simulink model "TestSupervisorFSM_RX"  (R2023b)
settings: Solver=FixedStepDiscrete  StartTime=0.0  StopTime=inf  FixedStep=0.001  RelTol=1e-3  EnableMultiTasking=on
model workspace (MAT data in the model file):
  Command = 1
  SelectedControlMode = 0
  State = 0
  pid_kp = 1
undefined symbols (not defined in the file): CANErrorTypes, ControlModes, MCControlModes
libraries: eeStairGenerator x7
settings Model: DataDictionary=EmbeddedBoardDD.sldd  Creator=vvasco  LastModifiedBy=upattacini
settings SolverCC: AlgebraicLoopSolver=TrustRegion  AutoInsertRateTranBlk=on
settings DataIOCC: LimitDataPoints=on
settings OptimizationCC: ReuseModelBlockBuffer=off  LifeSpan=inf
settings DebuggingCC: ParameterPrecisionLossMsg=none  UnconnectedInputMsg=warning  UnconnectedOutputMsg=warning  UnconnectedLineMsg=warning  AllowSymbolicDim=off  SFUnexpectedBacktrackingDiag=warning  SFNoUnconditionalDefaultTransitionDiag=warning  SFExecutionAtInitializationDiag=none  ArithmeticOperatorsInVariantConditions=warning
settings ModelReferenceCC: EnableRefExpFcnMdlSchedulingChecks=on
settings SFSimCC: SimUseLocalCustomCode=off  CustomCodeUndefinedFunction=UseInterfaceOnly
settings RTWCC: RTWUseLocalCustomCode=off  DLArmComputeVersion=19.05
settings CodeAppCC: StateflowObjectComments=on
settings GRTTargetCC: TargetLangStandard=C89/C90 (ANSI)
settings ConfigComp: CovMetricSettings=dw  CovSaveCumulativeToWorkspaceVar=on  CovSaveSingleToWorkspaceVar=on  CovExternalEMLEnable=off

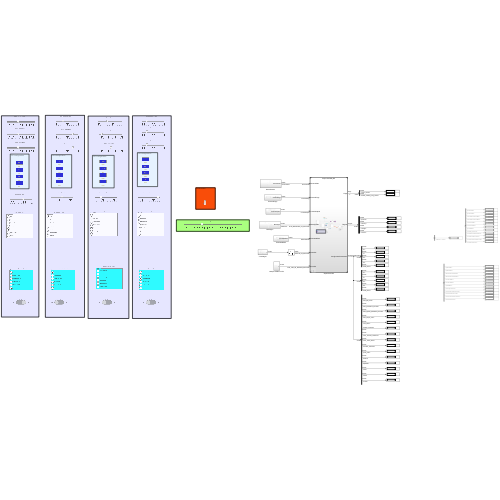
[thumbnail: Simulink's stored preview of the top-level diagram]
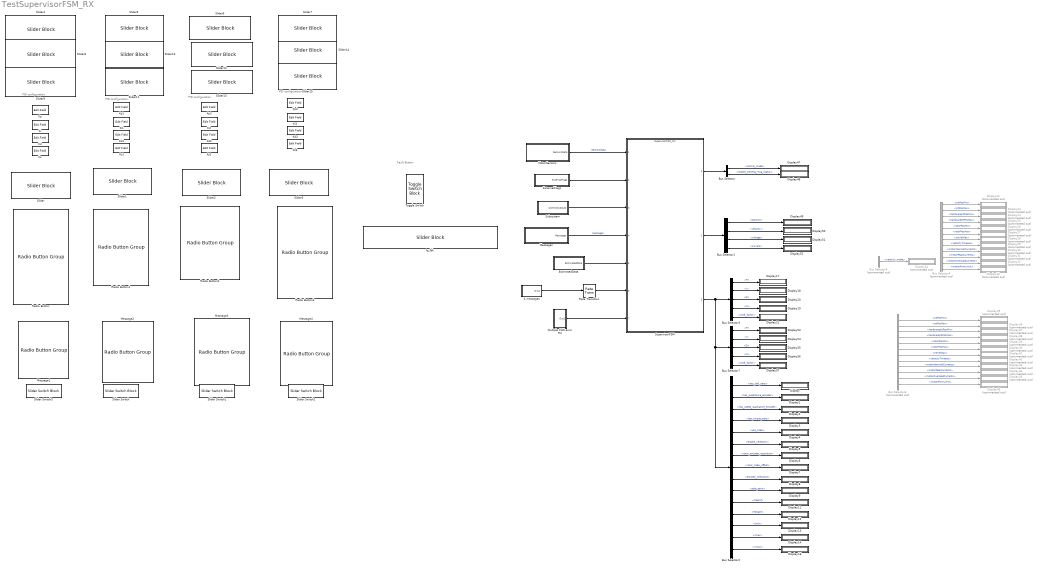
== system TestSupervisorFSM_RX ==
  note: Fault Button
  note: PID configuration
  note: PID configuration
  note: PID configuration
  note: PID configuration
  4 messages : Subsystem
  Bus Selector : BusSelector  OutputSignals=control_mode,enable_sending_msg_status
  Bus Selector1 : BusSelector  OutputSignals=jointpositions.position,jointvelocities.velocity,motorvoltage.voltage,motorcurrent.current
  Bus Selector2 : BusSelector  OutputSignals=motorconfig.has_hall_sens,motorconfig.has_quadrature_encoder,motorconfig.has_speed_quadrature_encoder,motorconfig.has_torque_sens,motorconfig.use_index,motorconfig.enable_verbosity,motorconfig.rotor_encoder_resolution,motorconfig.rotor_index_offset,motorconfig.encoder_tolerance,motorconfig.pole_pairs,motorconfig.Kbemf,motorconfig.Rphase,motorconfig.Imin,motorconfig.Imax,motorconfig.Vmax
  Bus Selector3 : BusSelector  OutputSignals=CurLoopPID.P,CurLoopPID.I,CurLoopPID.D,CurLoopPID.N,CurLoopPID.shift_factor
  Bus Selector4 : BusSelector  Commented=on  OutputSignals=thresholds.jntPosMin,thresholds.jntPosMax,thresholds.hardwareJntPosMin,thresholds.hardwareJntPosMax,thresholds.rotorPosMin,thresholds.rotorPosMax,thresholds.jntVelMax,thresholds.velocityTimeout,thresholds.motorNominalCurrents,thresholds.motorPeakCurrents,thresholds.motorOverloadCurrents,thresholds.motorPwmLimit
  Bus Selector5 : BusSelector  Commented=on  OutputSignals=estimationconfig.velocity_mode
  Bus Selector6 : BusSelector  Commented=on  OutputSignals=thresholds.jntPosMin,thresholds.jntPosMax,thresholds.hardwareJntPosMin,thresholds.hardwareJntPosMax,thresholds.rotorPosMin,thresholds.rotorPosMax,thresholds.jntVelMax,thresholds.velocityTimeout,thresholds.motorNominalCurrents,thresholds.motorPeakCurrents,thresholds.motorOverloadCurrents,thresholds.motorPwmLimit
  Bus Selector7 : BusSelector  OutputSignals=VelLoopPID.P,VelLoopPID.I,VelLoopPID.D,VelLoopPID.N,VelLoopPID.shift_factor
  Display{,1..9,11..14,16..21,47..57} (31 alike) : Display
  Display{22..46} (25 alike) : Display  Commented=on
  EstimatedData : Subsystem
  ExternalFlags : Subsystem
  Iq_fbk : SliderBlock  ScaleMax=20
  Kd{,1..3} (4 alike) : EditField  LabelPosition=Hide  ShowInitialText=on  Alignment=Center
  Ki{,1..3} (4 alike) : EditField  LabelPosition=Hide  ShowInitialText=on  Alignment=Center
  Kp{,1..3} (4 alike) : EditField  LabelPosition=Hide  ShowInitialText=on  Alignment=Center
  Ks{,1..3} (4 alike) : EditField  LabelPosition=Hide  ShowInitialText=on  Alignment=Center
  Message1 : RadioButtonGroup  SelectedLabel=Set MotorConfig  ButtonGroupName=Group
      settings: Values={{'Set control mode', 'Set current limits', 'Set desired targets', 'Set current PID', 'Set Velocity PID', 'Set MotorConfig'}, [0 1 2 3 4 5]}
  Message2 : RadioButtonGroup  SelectedLabel=Set control mode  ButtonGroupName=Group
      settings: Values={{'Set control mode', 'Set current limits', 'Set desired target', 'Set current PID', 'Set velocity PID', 'Set MotorConfig'}, [0 1 2 3 4 5]}
  Message3 : RadioButtonGroup  SelectedLabel=Set desired target  ButtonGroupName=Group
      settings: Values={{'Set control mode', 'Set current limits', 'Set desired target', 'Set current PID', 'Set velocity PID', 'Set MotorConfig'}, [0 1 2 3 4 5]}
  Message4 : RadioButtonGroup  SelectedLabel=Set desired target  ButtonGroupName=Group
      settings: Values={{'Set control mode', 'Set current limits', 'Set desired target', 'Set current PID', 'Set Velocity PID', 'Set MotorConfig'}, [0 1 2 3 4 5]}
  Messages : Subsystem
  MotorSensors : Subsystem
  Multiple CAN error RX : Subsystem
  Radio Button : RadioButtonGroup  SelectedLabel=Current  ButtonGroupName=Control Mode  UseEnumeratedDataType=on  EnumeratedDataType=MCControlModes
      settings: Values={{'Idle', 'OpenLoop', 'SpeedVoltage', 'SpeedCurrent', 'Current', 'NotConfigured', 'HWFault'}, [0 80 10 11 6 176 160]}
  Radio Button1 : RadioButtonGroup  SelectedLabel=Idle  ButtonGroupName=Control Mode  UseEnumeratedDataType=on  EnumeratedDataType=MCControlModes
      settings: Values={{'Idle', 'OpenLoop', 'SpeedVoltage', 'SpeedCurrent', 'Current', 'NotConfigured', 'HWFault'}, [0 80 10 11 6 176 160]}
  Radio Button2 : RadioButtonGroup  SelectedLabel=Current  ButtonGroupName=Control Mode  UseEnumeratedDataType=on  EnumeratedDataType=MCControlModes
      settings: Values={{'Idle', 'OpenLoop', 'SpeedVoltage', 'SpeedCurrent', 'Current', 'NotConfigured', 'HWFault'}, [0 80 10 11 6 176 160]}
  Radio Button3 : RadioButtonGroup  SelectedLabel=Current  ButtonGroupName=Control Mode  UseEnumeratedDataType=on  EnumeratedDataType=MCControlModes
      settings: Values={{'Idle', 'OpenLoop', 'SpeedVoltage', 'SpeedCurrent', 'Current', 'NotConfigured', 'HWFault'}, [0 80 10 11 6 176 160]}
  Rate Transition : RateTransition  Deterministic=off  OutPortSampleTimeOpt=Inherit
  Slider{,1..3} (4 alike) : SliderBlock  ScaleMin=10  ScaleMax=20
  Slider Switch{,1..3} (4 alike) : SliderSwitchBlock
      settings: Values={{'Off', 'On'}, [0 1]}
  Slider{4..15} (12 alike) : SliderBlock  ScaleMax=20
  Subsystem : Subsystem
  SupervisorFSM : ModelReference  ModelNameDialog=SupervisorFSM_RX.slx  SimulationMode=Normal  ModelReferenceVersion=7.4
  Toggle Switch : ToggleSwitchBlock  LabelPosition=Hide
      settings: Values={{'Off', 'On'}, [0 1]}
  wires:
  SupervisorFSM/2 -> Bus Selector1/1
  MotorSensors/1(SensorsData) -> SupervisorFSM/1  "SensorsData"
  SupervisorFSM/1 -> Bus Selector/1
  Bus Selector/1 -> Display47/1  "<control_mode>"
  Subsystem/1(ControlOutputs) -> SupervisorFSM/3
  ExternalFlags/1(externalFlags) -> SupervisorFSM/2
  Bus Selector/2 -> Display48/1  "<enable_sending_msg_status>"
  Bus Selector1/1 -> Display49/1  "<position>"
  Bus Selector1/2 -> Display50/1  "<velocity>"
  Bus Selector1/3 -> Display51/1  "<voltage>"
  Bus Selector1/4 -> Display52/1  "<current>"
  Rate Transition/1 -> SupervisorFSM/6
  Messages/1(Messages) -> SupervisorFSM/4  "Messages"
  EstimatedData/1(EstimatedData) -> SupervisorFSM/5
  Multiple CAN error RX/1(Out1) -> SupervisorFSM/7
  4 messages/1(Out1) -> Rate Transition/1
  Bus Selector2/1 -> Display/1  "<has_hall_sens>"
  Bus Selector2/2 -> Display1/1  "<has_quadrature_encoder>"
  Bus Selector2/3 -> Display2/1  "<has_speed_quadrature_encoder>"
  Bus Selector2/4 -> Display3/1  "<has_torque_sens>"
  Bus Selector2/5 -> Display4/1  "<use_index>"
  Bus Selector2/6 -> Display5/1  "<enable_verbosity>"
  Bus Selector2/7 -> Display6/1  "<rotor_encoder_resolution>"
  Bus Selector2/8 -> Display7/1  "<rotor_index_offset>"
  Bus Selector2/9 -> Display8/1  "<encoder_tolerance>"
  Bus Selector2/10 -> Display9/1  "<pole_pairs>"
  Bus Selector2/11 -> Display11/1  "<Kbemf>"
  Bus Selector2/12 -> Display12/1  "<Rphase>"
  Bus Selector2/13 -> Display13/1  "<Imin>"
  Bus Selector2/14 -> Display14/1  "<Imax>"
  Bus Selector3/1 -> Display17/1  "<P>"
  Bus Selector3/2 -> Display18/1  "<I>"
  Bus Selector3/3 -> Display20/1  "<D>"
  Bus Selector3/4 -> Display19/1  "<N>"
  Bus Selector3/5 -> Display21/1  "<shift_factor>"
  Bus Selector4/1 -> Display22/1  "<jntPosMin>"
  Bus Selector4/2 -> Display23/1  "<jntPosMax>"
  Bus Selector4/3 -> Display24/1  "<hardwareJntPosMin>"
  Bus Selector4/4 -> Display25/1  "<hardwareJntPosMax>"
  Bus Selector4/5 -> Display26/1  "<rotorPosMin>"
  Bus Selector4/6 -> Display27/1  "<rotorPosMax>"
  Bus Selector4/7 -> Display28/1  "<jntVelMax>"
  Bus Selector4/8 -> Display29/1  "<velocityTimeout>"
  Bus Selector4/9 -> Display30/1  "<motorNominalCurrents>"
  Bus Selector4/10 -> Display31/1  "<motorPeakCurrents>"
  Bus Selector4/11 -> Display32/1  "<motorOverloadCurrents>"
  Bus Selector4/12 -> Display33/1  "<motorPwmLimit>"
  Bus Selector5/1 -> Display34/1  "<velocity_mode>"
  Bus Selector6/1 -> Display35/1  "<jntPosMin>"
  Bus Selector6/2 -> Display36/1  "<jntPosMax>"
  Bus Selector6/3 -> Display37/1  "<hardwareJntPosMin>"
  Bus Selector6/4 -> Display38/1  "<hardwareJntPosMax>"
  Bus Selector6/5 -> Display39/1  "<rotorPosMin>"
  Bus Selector6/6 -> Display40/1  "<rotorPosMax>"
  Bus Selector6/7 -> Display41/1  "<jntVelMax>"
  Bus Selector6/8 -> Display42/1  "<velocityTimeout>"
  Bus Selector6/9 -> Display43/1  "<motorNominalCurrents>"
  Bus Selector6/10 -> Display44/1  "<motorPeakCurrents>"
  Bus Selector6/11 -> Display45/1  "<motorOverloadCurrents>"
  Bus Selector6/12 -> Display46/1  "<motorPwmLimit>"
  SupervisorFSM/3 -> Bus Selector2/1, Bus Selector7/1, Bus Selector3/1
  Bus Selector7/1 -> Display53/1  "<P>"
  Bus Selector7/2 -> Display54/1  "<I>"
  Bus Selector7/3 -> Display55/1  "<D>"
  Bus Selector7/4 -> Display56/1  "<N>"
  Bus Selector7/5 -> Display57/1  "<shift_factor>"
  Bus Selector2/15 -> Display16/1  "<Vmax>"

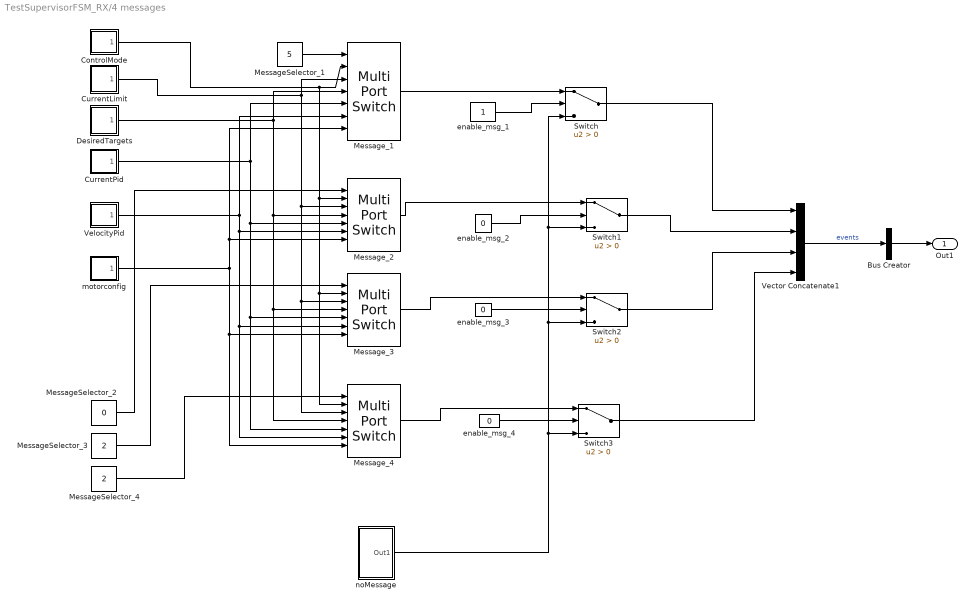
== system TestSupervisorFSM_RX/4 messages ==
  Bus Creator : BusCreator  Inputs=1  OutDataTypeStr=Bus: BUS_STATUS_RX_MULTIPLE  NonVirtualBus=on
      settings: InheritFromInputs=off
  ControlMode : Subsystem
  CurrentLimit : Subsystem
  CurrentPid : Subsystem
  DesiredTargets : Subsystem
  MessageSelector_1 : Constant  Value=5
  MessageSelector_2 : Constant  Value=0
  MessageSelector_3 : Constant  Value=2
  MessageSelector_4 : Constant  Value=2
  Message_{1..4} (4 alike) : MultiPortSwitch  DataPortOrder=Zero-based contiguous  Inputs=6  zeroidx=on  SaturateOnIntegerOverflow=off  InputSameDT=off
  Switch{,1..3} (4 alike) : Switch  Criteria=u2 > Threshold  SaturateOnIntegerOverflow=off  InputSameDT=off
  Vector Concatenate1 : Concatenate  NumInputs=4
  VelocityPid : Subsystem
  enable_msg_1 : Constant
  enable_msg_2 : Constant  Value=0
  enable_msg_3 : Constant  Value=0
  enable_msg_4 : Constant  Value=0
  motorconfig : Subsystem
  noMessage : Subsystem
  Out1 : Outport  OutDataTypeStr=Bus: BUS_STATUS_RX_MULTIPLE
  wires:
  MessageSelector_1/1 -> Message_1/1
  ControlMode/1(Out1) -> Message_4/2, Message_3/2, Message_2/2, Message_1/2
  CurrentPid/1(Out1) -> Message_2/5, Message_4/5, Message_3/5, Message_1/5
  MessageSelector_3/1 -> Message_3/1
  Vector Concatenate1/1 -> Bus Creator/1  "events"
  MessageSelector_4/1 -> Message_4/1
  DesiredTargets/1(Out1) -> Message_4/4, Message_3/4, Message_2/4, Message_1/4
  CurrentLimit/1(Out1) -> Message_4/3, Message_3/3, Message_2/3, Message_1/3
  MessageSelector_2/1 -> Message_2/1
  Bus Creator/1 -> Out1/1
  noMessage/1(Out1) -> Switch3/3, Switch1/3, Switch/3, Switch2/3
  enable_msg_1/1 -> Switch/2
  Message_1/1 -> Switch/1
  Message_2/1 -> Switch1/1
  enable_msg_2/1 -> Switch1/2
  Message_3/1 -> Switch2/1
  enable_msg_3/1 -> Switch2/2
  enable_msg_4/1 -> Switch3/2
  Message_4/1 -> Switch3/1
  Switch/1 -> Vector Concatenate1/1
  Switch1/1 -> Vector Concatenate1/2
  Switch2/1 -> Vector Concatenate1/3
  Switch3/1 -> Vector Concatenate1/4
  VelocityPid/1(Out1) -> Message_2/6, Message_4/6, Message_3/6, Message_1/6
  motorconfig/1(Out1) -> Message_4/7, Message_3/7, Message_2/7, Message_1/7

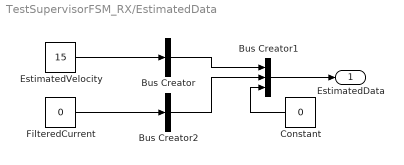
== system TestSupervisorFSM_RX/EstimatedData ==
  Bus Creator : BusCreator  Inputs=1  OutDataTypeStr=Bus: JointVelocities  NonVirtualBus=on
      settings: InheritFromInputs=off
  Bus Creator1 : BusCreator  Inputs=3  OutDataTypeStr=Bus: EstimatedData  NonVirtualBus=on
      settings: InheritFromInputs=off
  Bus Creator2 : BusCreator  Inputs=1  OutDataTypeStr=Bus: MotorCurrent  NonVirtualBus=on
      settings: InheritFromInputs=off
  Constant : Constant  Value=0  OutDataTypeStr=Bus: MotorTemperature
  EstimatedVelocity : Constant  Value=15  OutDataTypeStr=single
  FilteredCurrent : Constant  Value=0  OutDataTypeStr=single
  EstimatedData : Outport
  wires:
  EstimatedVelocity/1 -> Bus Creator/1
  Bus Creator1/1 -> EstimatedData/1
  Bus Creator/1 -> Bus Creator1/1
  FilteredCurrent/1 -> Bus Creator2/1
  Bus Creator2/1 -> Bus Creator1/2
  Constant/1 -> Bus Creator1/3

== system TestSupervisorFSM_RX/ExternalFlags ==
  Constant : Constant  Value=logical(0)  OutDataTypeStr=boolean
  ExternalFlags : BusCreator  Inputs=1  OutDataTypeStr=Bus: ExternalFlags
  externalFlags : Outport
  wires:
  Constant/1 -> ExternalFlags/1  "fault_button"
  ExternalFlags/1 -> externalFlags/1

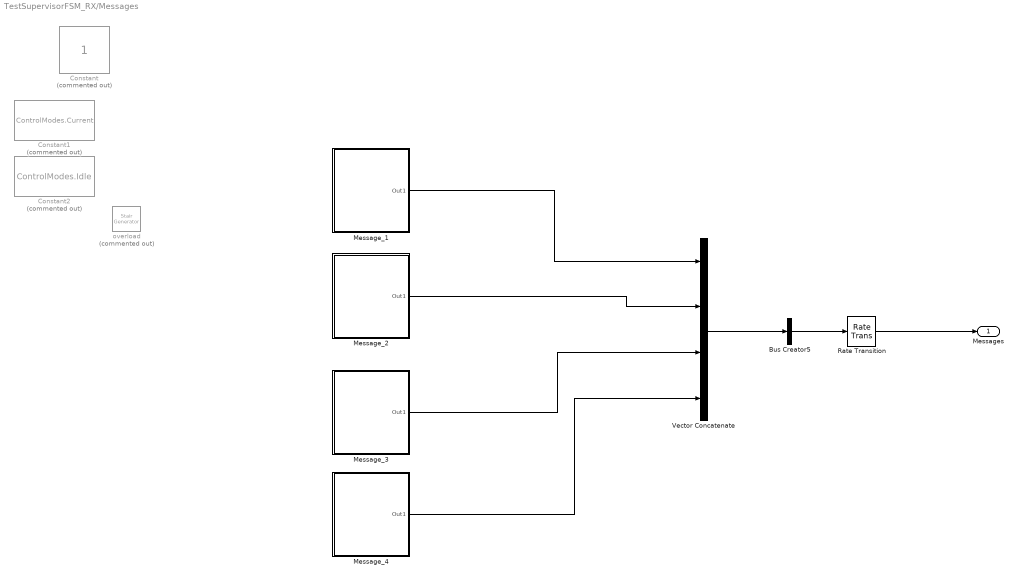
== system TestSupervisorFSM_RX/Messages ==
  Bus Creator5 : BusCreator  Inputs=1  OutDataTypeStr=Bus: BUS_MESSAGES_RX_MULTIPLE  NonVirtualBus=on
      settings: InheritFromInputs=off
  Constant : Constant  Commented=on  OutDataTypeStr=Enum: ControlModes
  Constant1 : Constant  Commented=on  Value=ControlModes.Current  OutDataTypeStr=Enum: ControlModes
  Constant2 : Constant  Commented=on  Value=ControlModes.Idle  OutDataTypeStr=Enum: ControlModes
  Message_1 : Subsystem
  Message_2 : Subsystem
  Message_3 : Subsystem
  Message_4 : Subsystem
  Rate Transition : RateTransition  Deterministic=off  OutPortSampleTimeOpt=Inherit
  Vector Concatenate : Concatenate  NumInputs=4
  overload : eeStairGenerator/Stair Generator  Commented=on  LabelModeActiveChoice=Discrete  TimeInput=[0 0.1 0.2 0.3 0.4 0.5 0.6 0.7 0.8 0.9]  AmplitudeInput=[5 0 5 1 1 1 1 1 1 1]  SampleTime=0.1  RepeatPattern=off  OutDataTypeStr=uint16
  Messages : Outport
  wires:
  Rate Transition/1 -> Messages/1
  Vector Concatenate/1 -> Bus Creator5/1
  Message_1/1(Out1) -> Vector Concatenate/1
  Message_2/1(Out1) -> Vector Concatenate/2
  Message_3/1(Out1) -> Vector Concatenate/3
  Message_4/1(Out1) -> Vector Concatenate/4
  Bus Creator5/1 -> Rate Transition/1

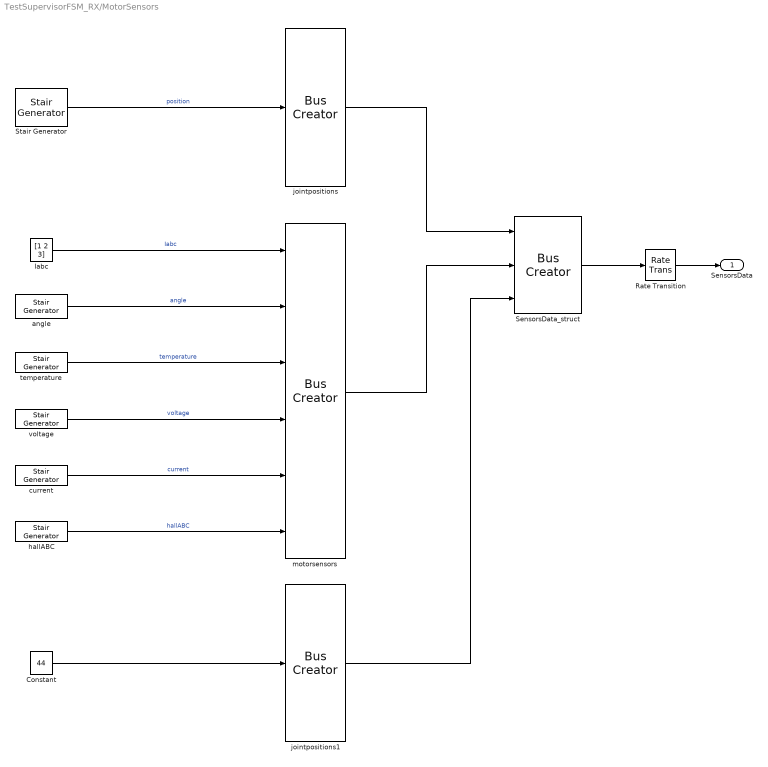
== system TestSupervisorFSM_RX/MotorSensors ==
  Constant : Constant  Value=44  OutDataTypeStr=single
  Iabc : Constant  Value=[1 2 3]  OutDataTypeStr=single
  Rate Transition : RateTransition  Deterministic=off  OutPortSampleTimeOpt=Inherit
  SensorsData_struct : BusCreator  Inputs=3  OutDataTypeStr=Bus: SensorsData
      settings: InheritFromInputs=off
  Stair Generator : eeStairGenerator/Stair Generator  LabelModeActiveChoice=Discrete  TimeInput=[0.1 0.2 0.3 0.4 0.5 0.6 0.7 0.8 0.9 1 1.1 1.2 1.3 ]  AmplitudeInput=[20 23 26 29 32 35 38 41 39 36 30 25 20]  SampleTime=0.1  RepeatPattern=on  OutDataTypeStr=single
  angle : eeStairGenerator/Stair Generator  LabelModeActiveChoice=Discrete  TimeInput=[0 1 2 3 4 5 6 7 8 9]  AmplitudeInput=[0 1 6 6 6 1 1 1 2 2]  SampleTime=0.1  RepeatPattern=off  OutDataTypeStr=single
  current : eeStairGenerator/Stair Generator  LabelModeActiveChoice=Discrete  TimeInput=[0 0.1 0.2 0.3 0.4 0.5 0.6 0.7 0.8 0.9]  AmplitudeInput=[16 10 15 12 10 16 12 16 18 17]  SampleTime=0.1  RepeatPattern=on  OutDataTypeStr=single
  hallABC : eeStairGenerator/Stair Generator  LabelModeActiveChoice=Discrete  TimeInput=[0 0.1 0.2 0.3 0.4 0.5 0.6 0.7 0.8 0.9]  AmplitudeInput=[6 3 5 2 0 6 6 6 6 6]  SampleTime=0.1  RepeatPattern=off  OutDataTypeStr=uint8
  jointpositions : BusCreator  Inputs=1  OutDataTypeStr=Bus: JointPositions
      settings: InheritFromInputs=off
  jointpositions1 : BusCreator  Inputs=1  OutDataTypeStr=Bus: SupplyVoltage
      settings: InheritFromInputs=off
  motorsensors : BusCreator  Inputs=6  OutDataTypeStr=Bus: MotorSensors
      settings: InheritFromInputs=off
  temperature : eeStairGenerator/Stair Generator  LabelModeActiveChoice=Discrete  TimeInput=[0 1 2 3 4 5 6 7 8 9]  AmplitudeInput=[2 2 2 9 9 9 9 9 9 2]  SampleTime=0.1  RepeatPattern=off  OutDataTypeStr=single
  voltage : eeStairGenerator/Stair Generator  LabelModeActiveChoice=Discrete  TimeInput=[0 1 2 3 4 5 6 7 8 9]./10  AmplitudeInput=[2 3 3 3 3 3 2 2 2 2]  SampleTime=0.1  RepeatPattern=on  OutDataTypeStr=single
  SensorsData : Outport  OutDataTypeStr=Bus: SensorsData
  wires:
  motorsensors/1 -> SensorsData_struct/2
  voltage/1 -> motorsensors/4  "voltage"
  angle/1 -> motorsensors/2  "angle"
  temperature/1 -> motorsensors/3  "temperature"
  current/1 -> motorsensors/5  "current"
  Iabc/1 -> motorsensors/1  "Iabc"
  hallABC/1 -> motorsensors/6  "hallABC"
  SensorsData_struct/1 -> Rate Transition/1
  Stair Generator/1 -> jointpositions/1  "position"
  jointpositions/1 -> SensorsData_struct/1
  Rate Transition/1 -> SensorsData/1
  jointpositions1/1 -> SensorsData_struct/3
  Constant/1 -> jointpositions1/1

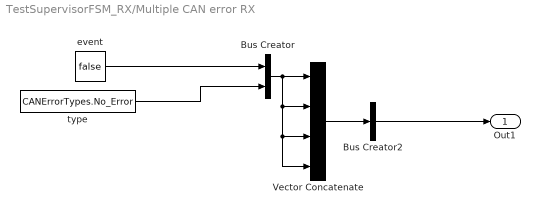
== system TestSupervisorFSM_RX/Multiple CAN error RX ==
  Bus Creator : BusCreator  Inputs=2  OutDataTypeStr=Bus: BUS_CAN_RX_ERRORS  NonVirtualBus=on
      settings: InheritFromInputs=off
  Bus Creator2 : BusCreator  Inputs=1  OutDataTypeStr=Bus: BUS_CAN_RX_ERRORS_MULTIPLE  NonVirtualBus=on
      settings: InheritFromInputs=off
  Vector Concatenate : Concatenate  NumInputs=4
  event : Constant  Value=false  OutDataTypeStr=boolean
  type : Constant  Value=CANErrorTypes.No_Error  OutDataTypeStr=Enum: CANErrorTypes
  Out1 : Outport
  wires:
  Bus Creator/1 -> Vector Concatenate/4, Vector Concatenate/3, Vector Concatenate/2, Vector Concatenate/1
  event/1 -> Bus Creator/1
  type/1 -> Bus Creator/2
  Vector Concatenate/1 -> Bus Creator2/1
  Bus Creator2/1 -> Out1/1

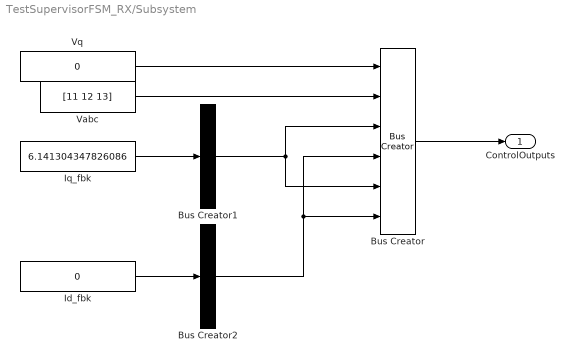
== system TestSupervisorFSM_RX/Subsystem ==
  Bus Creator : BusCreator  Inputs=6  OutDataTypeStr=Bus: ControlOutputs
      settings: InheritFromInputs=off
  Bus Creator1 : BusCreator  Inputs=1  OutDataTypeStr=Bus: MotorCurrent
      settings: InheritFromInputs=off
  Bus Creator2 : BusCreator  Inputs=1  OutDataTypeStr=Bus: MotorCurrent
      settings: InheritFromInputs=off
  Id_fbk : Constant  Value=0  OutDataTypeStr=single
  Iq_fbk : Constant  Value=6.141304347826086  OutDataTypeStr=single
  Vabc : Constant  Value=[11 12 13]  OutDataTypeStr=single
  Vq : Constant  Value=0  OutDataTypeStr=single
  ControlOutputs : Outport  OutDataTypeStr=Bus: ControlOutputs
  wires:
  Iq_fbk/1 -> Bus Creator1/1
  Bus Creator/1 -> ControlOutputs/1
  Bus Creator1/1 -> Bus Creator/5, Bus Creator/3
  Vabc/1 -> Bus Creator/2
  Vq/1 -> Bus Creator/1
  Bus Creator2/1 -> Bus Creator/6, Bus Creator/4
  Id_fbk/1 -> Bus Creator2/1

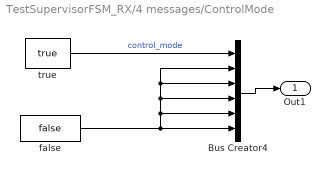
== system TestSupervisorFSM_RX/4 messages/ControlMode ==
  Bus Creator4 : BusCreator  Inputs=6  OutDataTypeStr=Bus: BUS_STATUS_RX  NonVirtualBus=on
      settings: InheritFromInputs=off
  false : Constant  Value=false  OutDataTypeStr=boolean
  true : Constant  Value=true  OutDataTypeStr=boolean
  Out1 : Outport  OutDataTypeStr=Bus: BUS_STATUS_RX
  wires:
  true/1 -> Bus Creator4/1  "control_mode"
  false/1 -> Bus Creator4/6, Bus Creator4/2, Bus Creator4/3, Bus Creator4/4, Bus Creator4/5
  Bus Creator4/1 -> Out1/1

== system TestSupervisorFSM_RX/4 messages/CurrentLimit ==
  Bus Creator5 : BusCreator  Inputs=6  OutDataTypeStr=Bus: BUS_STATUS_RX  NonVirtualBus=on
      settings: InheritFromInputs=off
  false1 : Constant  Value=false  OutDataTypeStr=boolean
  true1 : Constant  Value=true  OutDataTypeStr=boolean
  Out1 : Outport  OutDataTypeStr=Bus: BUS_STATUS_RX
  wires:
  false1/1 -> Bus Creator5/6, Bus Creator5/5, Bus Creator5/1, Bus Creator5/3, Bus Creator5/4
  true1/1 -> Bus Creator5/2
  Bus Creator5/1 -> Out1/1

== system TestSupervisorFSM_RX/4 messages/CurrentPid ==
  Bus Creator7 : BusCreator  Inputs=6  OutDataTypeStr=Bus: BUS_STATUS_RX  NonVirtualBus=on
      settings: InheritFromInputs=off
  false3 : Constant  Value=false  OutDataTypeStr=boolean
  true3 : Constant  Value=true  OutDataTypeStr=boolean
  Out1 : Outport  OutDataTypeStr=Bus: BUS_STATUS_RX
  wires:
  true3/1 -> Bus Creator7/4  "control_mode"
  false3/1 -> Bus Creator7/6, Bus Creator7/5, Bus Creator7/3, Bus Creator7/2, Bus Creator7/1
  Bus Creator7/1 -> Out1/1

== system TestSupervisorFSM_RX/4 messages/DesiredTargets ==
  Bus Creator6 : BusCreator  Inputs=6  OutDataTypeStr=Bus: BUS_STATUS_RX  NonVirtualBus=on
      settings: InheritFromInputs=off
  false2 : Constant  Value=false  OutDataTypeStr=boolean
  true2 : Constant  Value=true  OutDataTypeStr=boolean
  Out1 : Outport  OutDataTypeStr=Bus: BUS_STATUS_RX
  wires:
  true2/1 -> Bus Creator6/3  "control_mode"
  false2/1 -> Bus Creator6/6, Bus Creator6/5, Bus Creator6/2, Bus Creator6/1, Bus Creator6/4
  Bus Creator6/1 -> Out1/1

== system TestSupervisorFSM_RX/4 messages/VelocityPid ==
  Bus Creator7 : BusCreator  Inputs=6  OutDataTypeStr=Bus: BUS_STATUS_RX  NonVirtualBus=on
      settings: InheritFromInputs=off
  false3 : Constant  Value=false  OutDataTypeStr=boolean
  true3 : Constant  Value=true  OutDataTypeStr=boolean
  Out1 : Outport  OutDataTypeStr=Bus: BUS_STATUS_RX
  wires:
  true3/1 -> Bus Creator7/5  "control_mode"
  false3/1 -> Bus Creator7/3, Bus Creator7/6, Bus Creator7/4, Bus Creator7/2, Bus Creator7/1
  Bus Creator7/1 -> Out1/1

== system TestSupervisorFSM_RX/4 messages/motorconfig ==
  Bus Creator7 : BusCreator  Inputs=6  OutDataTypeStr=Bus: BUS_STATUS_RX  NonVirtualBus=on
      settings: InheritFromInputs=off
  false3 : Constant  Value=false  OutDataTypeStr=boolean
  true3 : Constant  Value=true  OutDataTypeStr=boolean
  Out1 : Outport  OutDataTypeStr=Bus: BUS_STATUS_RX
  wires:
  true3/1 -> Bus Creator7/6  "control_mode"
  false3/1 -> Bus Creator7/3, Bus Creator7/5, Bus Creator7/4, Bus Creator7/2, Bus Creator7/1
  Bus Creator7/1 -> Out1/1

== system TestSupervisorFSM_RX/4 messages/noMessage ==
  Bus Creator : BusCreator  Inputs=6  OutDataTypeStr=Bus: BUS_STATUS_RX  NonVirtualBus=on
      settings: InheritFromInputs=off
  Constant : Constant  Value=false
  Out1 : Outport
  wires:
  Constant/1 -> Bus Creator/6, Bus Creator/5, Bus Creator/4, Bus Creator/3, Bus Creator/2, Bus Creator/1
  Bus Creator/1 -> Out1/1

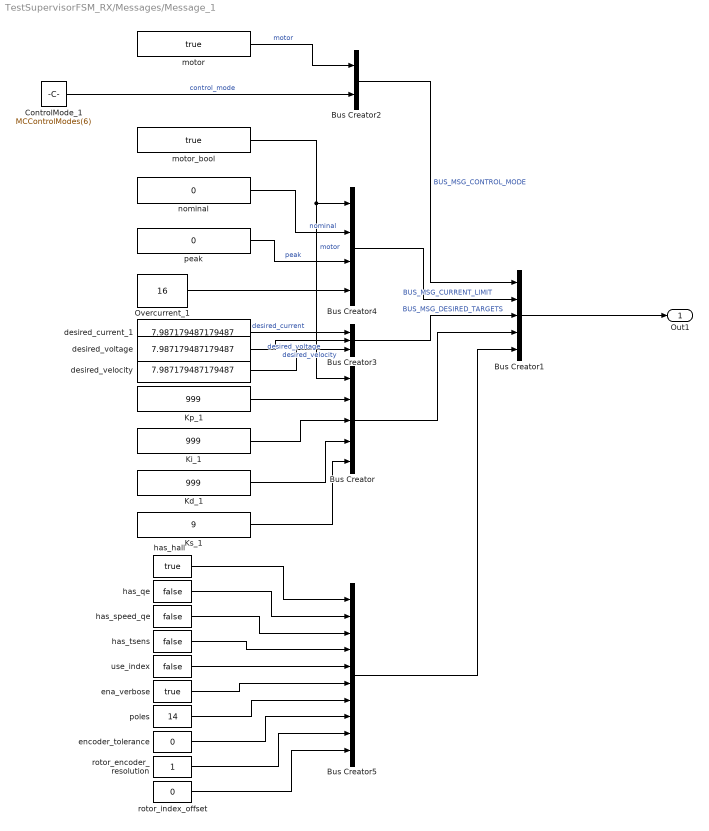
== system TestSupervisorFSM_RX/Messages/Message_1 ==
  Bus Creator : BusCreator  Inputs=5  OutDataTypeStr=Bus: BUS_MSG_PID  NonVirtualBus=on
      settings: InheritFromInputs=off
  Bus Creator1 : BusCreator  Inputs=5  OutDataTypeStr=Bus: BUS_MESSAGES_RX  NonVirtualBus=on
      settings: InheritFromInputs=off
  Bus Creator2 : BusCreator  Inputs=2  OutDataTypeStr=Bus: BUS_MSG_CONTROL_MODE  NonVirtualBus=on
      settings: InheritFromInputs=off
  Bus Creator3 : BusCreator  Inputs=3  OutDataTypeStr=Bus: BUS_MSG_DESIRED_TARGETS  NonVirtualBus=on
      settings: InheritFromInputs=off
  Bus Creator4 : BusCreator  Inputs=4  OutDataTypeStr=Bus: BUS_MSG_CURRENT_LIMIT  NonVirtualBus=on
      settings: InheritFromInputs=off
  Bus Creator5 : BusCreator  Inputs=10  OutDataTypeStr=Bus: BUS_MSG_MOTOR_CONFIG  NonVirtualBus=on
      settings: InheritFromInputs=off
  ControlMode_1 : Constant  Value=MCControlModes(6)  OutDataTypeStr=Enum: MCControlModes
  Kd_1 : Constant  Value=999  OutDataTypeStr=single
  Ki_1 : Constant  Value=999  OutDataTypeStr=single
  Kp_1 : Constant  Value=999  OutDataTypeStr=single
  Ks_1 : Constant  Value=9  OutDataTypeStr=uint8
  Overcurrent_1 : Constant  Value=16  OutDataTypeStr=single
  desired_current_1 : Constant  Value=7.987179487179487  OutDataTypeStr=single
  desired_velocity : Constant  Value=7.987179487179487  OutDataTypeStr=single
  desired_voltage : Constant  Value=7.987179487179487  OutDataTypeStr=single
  ena_verbose : Constant  Value=true  OutDataTypeStr=boolean
  encoder_tolerance : Constant  Value=0  OutDataTypeStr=uint8
  has_hall : Constant  Value=true  OutDataTypeStr=boolean
  has_qe : Constant  Value=false  OutDataTypeStr=boolean
  has_speed_qe : Constant  Value=false  OutDataTypeStr=boolean
  has_tsens : Constant  Value=false  OutDataTypeStr=boolean
  motor : Constant  Value=true  OutDataTypeStr=boolean
  motor_bool : Constant  Value=true  OutDataTypeStr=boolean
  nominal : Constant  Value=0  OutDataTypeStr=single
  peak : Constant  Value=0  OutDataTypeStr=single
  poles : Constant  Value=14  OutDataTypeStr=uint8
  rotor_encoder_resolution : Constant  OutDataTypeStr=int16
  rotor_index_offset : Constant  Value=0  OutDataTypeStr=int16
  use_index : Constant  Value=false  OutDataTypeStr=boolean
  Out1 : Outport
  wires:
  desired_current_1/1 -> Bus Creator3/1  "desired_current"
  motor_bool/1 -> Bus Creator/1, Bus Creator4/1  "motor"
  Bus Creator3/1 -> Bus Creator1/3  "BUS_MSG_DESIRED_TARGETS"
  Bus Creator2/1 -> Bus Creator1/1  "BUS_MSG_CONTROL_MODE"
  motor/1 -> Bus Creator2/1  "motor"
  Bus Creator/1 -> Bus Creator1/4
  Kp_1/1 -> Bus Creator/2
  Ki_1/1 -> Bus Creator/3
  peak/1 -> Bus Creator4/3  "peak"
  nominal/1 -> Bus Creator4/2  "nominal"
  Bus Creator4/1 -> Bus Creator1/2  "BUS_MSG_CURRENT_LIMIT"
  Overcurrent_1/1 -> Bus Creator4/4
  Ks_1/1 -> Bus Creator/5
  Kd_1/1 -> Bus Creator/4
  ControlMode_1/1 -> Bus Creator2/2  "control_mode"
  Bus Creator1/1 -> Out1/1
  use_index/1 -> Bus Creator5/5
  has_tsens/1 -> Bus Creator5/4
  ena_verbose/1 -> Bus Creator5/6
  has_speed_qe/1 -> Bus Creator5/3
  poles/1 -> Bus Creator5/7
  has_qe/1 -> Bus Creator5/2
  encoder_tolerance/1 -> Bus Creator5/8
  has_hall/1 -> Bus Creator5/1
  rotor_encoder_resolution/1 -> Bus Creator5/9
  rotor_index_offset/1 -> Bus Creator5/10
  Bus Creator5/1 -> Bus Creator1/5
  desired_voltage/1 -> Bus Creator3/2  "desired_voltage"
  desired_velocity/1 -> Bus Creator3/3  "desired_velocity"

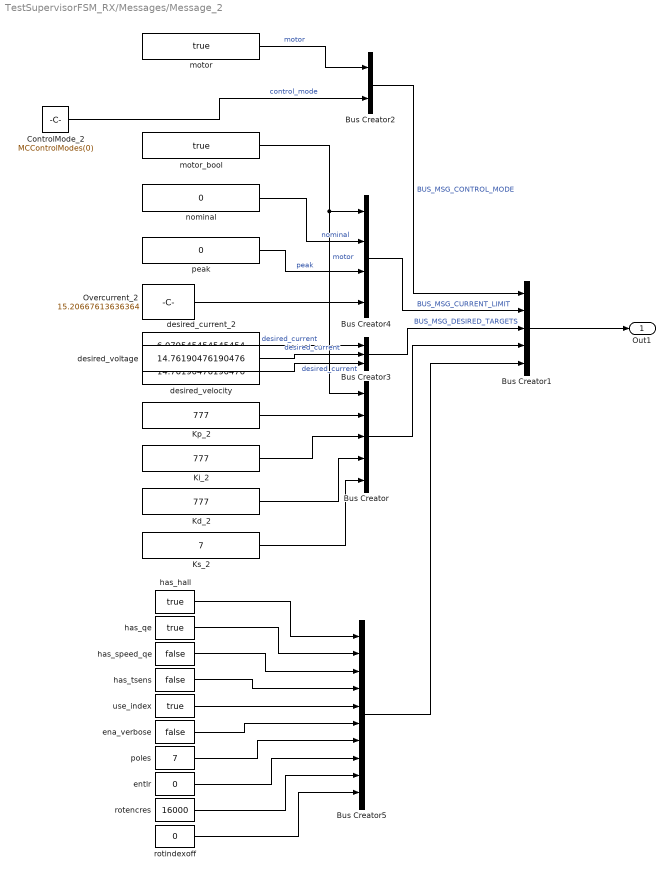
== system TestSupervisorFSM_RX/Messages/Message_2 ==
  Bus Creator : BusCreator  Inputs=5  OutDataTypeStr=Bus: BUS_MSG_PID  NonVirtualBus=on
      settings: InheritFromInputs=off
  Bus Creator1 : BusCreator  Inputs=5  OutDataTypeStr=Bus: BUS_MESSAGES_RX  NonVirtualBus=on
      settings: InheritFromInputs=off
  Bus Creator2 : BusCreator  Inputs=2  OutDataTypeStr=Bus: BUS_MSG_CONTROL_MODE  NonVirtualBus=on
      settings: InheritFromInputs=off
  Bus Creator3 : BusCreator  Inputs=3  OutDataTypeStr=Bus: BUS_MSG_DESIRED_TARGETS  NonVirtualBus=on
      settings: InheritFromInputs=off
  Bus Creator4 : BusCreator  Inputs=4  OutDataTypeStr=Bus: BUS_MSG_CURRENT_LIMIT  NonVirtualBus=on
      settings: InheritFromInputs=off
  Bus Creator5 : BusCreator  Inputs=10  OutDataTypeStr=Bus: BUS_MSG_MOTOR_CONFIG  NonVirtualBus=on
      settings: InheritFromInputs=off
  ControlMode_2 : Constant  Value=MCControlModes(0)  OutDataTypeStr=Enum: MCControlModes
  Kd_2 : Constant  Value=777  OutDataTypeStr=single
  Ki_2 : Constant  Value=777  OutDataTypeStr=single
  Kp_2 : Constant  Value=777  OutDataTypeStr=single
  Ks_2 : Constant  Value=7  OutDataTypeStr=uint8
  Overcurrent_2 : Constant  Value=15.20667613636364  OutDataTypeStr=single
  desired_current_2 : Constant  Value=6.079545454545454  OutDataTypeStr=single
  desired_velocity : Constant  Value=14.76190476190476  OutDataTypeStr=single
  desired_voltage : Constant  Value=14.76190476190476  OutDataTypeStr=single
  ena_verbose : Constant  Value=false  OutDataTypeStr=boolean
  entlr : Constant  Value=0  OutDataTypeStr=uint8
  has_hall : Constant  Value=true  OutDataTypeStr=boolean
  has_qe : Constant  Value=true  OutDataTypeStr=boolean
  has_speed_qe : Constant  Value=false  OutDataTypeStr=boolean
  has_tsens : Constant  Value=false  OutDataTypeStr=boolean
  motor : Constant  Value=true  OutDataTypeStr=boolean
  motor_bool : Constant  Value=true  OutDataTypeStr=boolean
  nominal : Constant  Value=0  OutDataTypeStr=single
  peak : Constant  Value=0  OutDataTypeStr=single
  poles : Constant  Value=7  OutDataTypeStr=uint8
  rotencres : Constant  Value=16000  OutDataTypeStr=int16
  rotindexoff : Constant  Value=0  OutDataTypeStr=int16
  use_index : Constant  Value=true  OutDataTypeStr=boolean
  Out1 : Outport
  wires:
  desired_current_2/1 -> Bus Creator3/1  "desired_current"
  motor_bool/1 -> Bus Creator/1, Bus Creator4/1  "motor"
  Bus Creator3/1 -> Bus Creator1/3  "BUS_MSG_DESIRED_TARGETS"
  Bus Creator2/1 -> Bus Creator1/1  "BUS_MSG_CONTROL_MODE"
  motor/1 -> Bus Creator2/1  "motor"
  Bus Creator/1 -> Bus Creator1/4
  Kp_2/1 -> Bus Creator/2
  Ki_2/1 -> Bus Creator/3
  peak/1 -> Bus Creator4/3  "peak"
  nominal/1 -> Bus Creator4/2  "nominal"
  Bus Creator4/1 -> Bus Creator1/2  "BUS_MSG_CURRENT_LIMIT"
  Overcurrent_2/1 -> Bus Creator4/4
  Ks_2/1 -> Bus Creator/5
  Kd_2/1 -> Bus Creator/4
  ControlMode_2/1 -> Bus Creator2/2  "control_mode"
  Bus Creator1/1 -> Out1/1
  rotindexoff/1 -> Bus Creator5/10
  rotencres/1 -> Bus Creator5/9
  entlr/1 -> Bus Creator5/8
  has_tsens/1 -> Bus Creator5/4
  ena_verbose/1 -> Bus Creator5/6
  use_index/1 -> Bus Creator5/5
  poles/1 -> Bus Creator5/7
  has_speed_qe/1 -> Bus Creator5/3
  has_qe/1 -> Bus Creator5/2
  has_hall/1 -> Bus Creator5/1
  Bus Creator5/1 -> Bus Creator1/5
  desired_voltage/1 -> Bus Creator3/2  "desired_current"
  desired_velocity/1 -> Bus Creator3/3  "desired_current"

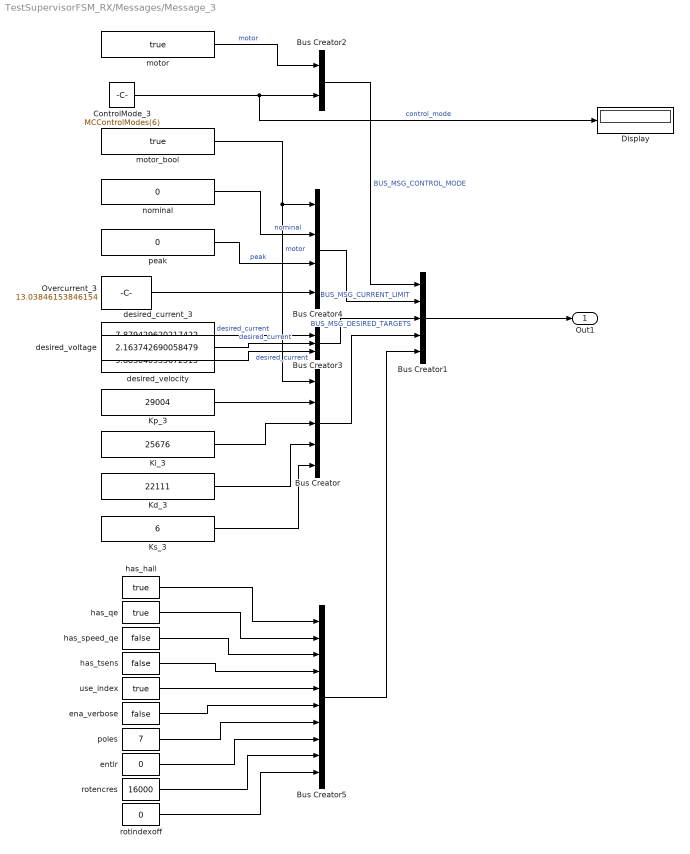
== system TestSupervisorFSM_RX/Messages/Message_3 ==
  Bus Creator : BusCreator  Inputs=5  OutDataTypeStr=Bus: BUS_MSG_PID  NonVirtualBus=on
      settings: InheritFromInputs=off
  Bus Creator1 : BusCreator  Inputs=5  OutDataTypeStr=Bus: BUS_MESSAGES_RX  NonVirtualBus=on
      settings: InheritFromInputs=off
  Bus Creator2 : BusCreator  Inputs=2  OutDataTypeStr=Bus: BUS_MSG_CONTROL_MODE  NonVirtualBus=on
      settings: InheritFromInputs=off
  Bus Creator3 : BusCreator  Inputs=3  OutDataTypeStr=Bus: BUS_MSG_DESIRED_TARGETS  NonVirtualBus=on
      settings: InheritFromInputs=off
  Bus Creator4 : BusCreator  Inputs=4  OutDataTypeStr=Bus: BUS_MSG_CURRENT_LIMIT  NonVirtualBus=on
      settings: InheritFromInputs=off
  Bus Creator5 : BusCreator  Inputs=10  OutDataTypeStr=Bus: BUS_MSG_MOTOR_CONFIG  NonVirtualBus=on
      settings: InheritFromInputs=off
  ControlMode_3 : Constant  Value=MCControlModes(6)  OutDataTypeStr=Enum: MCControlModes
  Display : Display
  Kd_3 : Constant  Value=22111  OutDataTypeStr=single
  Ki_3 : Constant  Value=25676  OutDataTypeStr=single
  Kp_3 : Constant  Value=29004  OutDataTypeStr=single
  Ks_3 : Constant  Value=6  OutDataTypeStr=uint8
  Overcurrent_3 : Constant  Value=13.03846153846154  OutDataTypeStr=single
  desired_current_3 : Constant  Value=7.879429620217422  OutDataTypeStr=single
  desired_velocity : Constant  Value=9.883040935672515  OutDataTypeStr=single
  desired_voltage : Constant  Value=2.163742690058479  OutDataTypeStr=single
  ena_verbose : Constant  Value=false  OutDataTypeStr=boolean
  entlr : Constant  Value=0  OutDataTypeStr=uint8
  has_hall : Constant  Value=true  OutDataTypeStr=boolean
  has_qe : Constant  Value=true  OutDataTypeStr=boolean
  has_speed_qe : Constant  Value=false  OutDataTypeStr=boolean
  has_tsens : Constant  Value=false  OutDataTypeStr=boolean
  motor : Constant  Value=true  OutDataTypeStr=boolean
  motor_bool : Constant  Value=true  OutDataTypeStr=boolean
  nominal : Constant  Value=0  OutDataTypeStr=single
  peak : Constant  Value=0  OutDataTypeStr=single
  poles : Constant  Value=7  OutDataTypeStr=uint8
  rotencres : Constant  Value=16000  OutDataTypeStr=int16
  rotindexoff : Constant  Value=0  OutDataTypeStr=int16
  use_index : Constant  Value=true  OutDataTypeStr=boolean
  Out1 : Outport
  wires:
  desired_current_3/1 -> Bus Creator3/1  "desired_current"
  motor_bool/1 -> Bus Creator/1, Bus Creator4/1  "motor"
  Bus Creator3/1 -> Bus Creator1/3  "BUS_MSG_DESIRED_TARGETS"
  Bus Creator2/1 -> Bus Creator1/1  "BUS_MSG_CONTROL_MODE"
  motor/1 -> Bus Creator2/1  "motor"
  Bus Creator/1 -> Bus Creator1/4
  Kp_3/1 -> Bus Creator/2
  Ki_3/1 -> Bus Creator/3
  peak/1 -> Bus Creator4/3  "peak"
  nominal/1 -> Bus Creator4/2  "nominal"
  Bus Creator4/1 -> Bus Creator1/2  "BUS_MSG_CURRENT_LIMIT"
  Overcurrent_3/1 -> Bus Creator4/4
  Ks_3/1 -> Bus Creator/5
  Kd_3/1 -> Bus Creator/4
  ControlMode_3/1 -> Display/1, Bus Creator2/2  "control_mode"
  Bus Creator1/1 -> Out1/1
  has_speed_qe/1 -> Bus Creator5/3
  has_hall/1 -> Bus Creator5/1
  rotindexoff/1 -> Bus Creator5/10
  entlr/1 -> Bus Creator5/8
  has_tsens/1 -> Bus Creator5/4
  rotencres/1 -> Bus Creator5/9
  poles/1 -> Bus Creator5/7
  ena_verbose/1 -> Bus Creator5/6
  has_qe/1 -> Bus Creator5/2
  use_index/1 -> Bus Creator5/5
  Bus Creator5/1 -> Bus Creator1/5
  desired_voltage/1 -> Bus Creator3/2  "desired_current"
  desired_velocity/1 -> Bus Creator3/3  "desired_current"

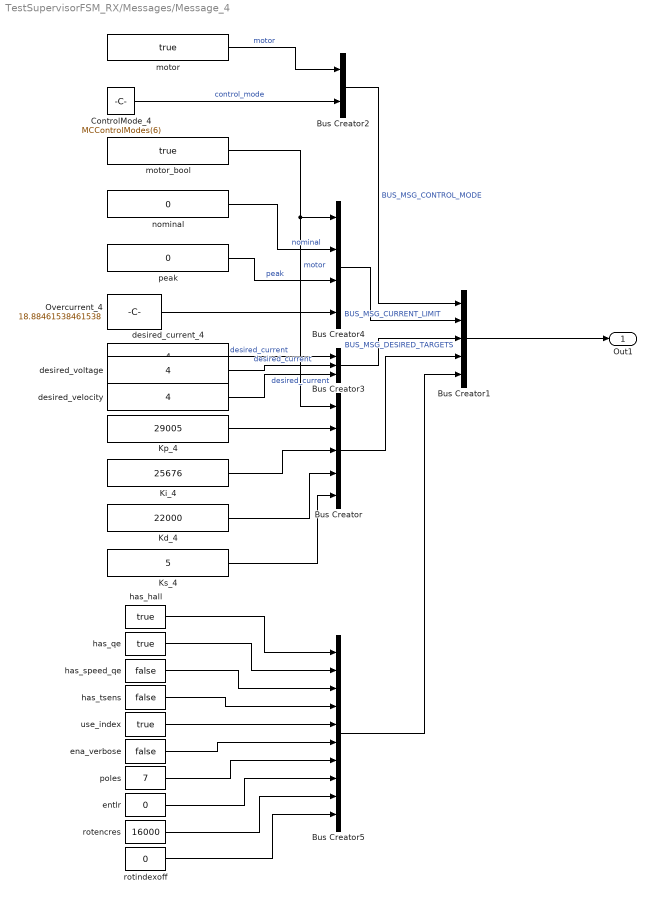
== system TestSupervisorFSM_RX/Messages/Message_4 ==
  Bus Creator : BusCreator  Inputs=5  OutDataTypeStr=Bus: BUS_MSG_PID  NonVirtualBus=on
      settings: InheritFromInputs=off
  Bus Creator1 : BusCreator  Inputs=5  OutDataTypeStr=Bus: BUS_MESSAGES_RX  NonVirtualBus=on
      settings: InheritFromInputs=off
  Bus Creator2 : BusCreator  Inputs=2  OutDataTypeStr=Bus: BUS_MSG_CONTROL_MODE  NonVirtualBus=on
      settings: InheritFromInputs=off
  Bus Creator3 : BusCreator  Inputs=3  OutDataTypeStr=Bus: BUS_MSG_DESIRED_TARGETS  NonVirtualBus=on
      settings: InheritFromInputs=off
  Bus Creator4 : BusCreator  Inputs=4  OutDataTypeStr=Bus: BUS_MSG_CURRENT_LIMIT  NonVirtualBus=on
      settings: InheritFromInputs=off
  Bus Creator5 : BusCreator  Inputs=10  OutDataTypeStr=Bus: BUS_MSG_MOTOR_CONFIG  NonVirtualBus=on
      settings: InheritFromInputs=off
  ControlMode_4 : Constant  Value=MCControlModes(6)  OutDataTypeStr=Enum: MCControlModes
  Kd_4 : Constant  Value=22000  OutDataTypeStr=single
  Ki_4 : Constant  Value=25676  OutDataTypeStr=single
  Kp_4 : Constant  Value=29005  OutDataTypeStr=single
  Ks_4 : Constant  Value=5  OutDataTypeStr=uint8
  Overcurrent_4 : Constant  Value=18.88461538461538  OutDataTypeStr=single
  desired_current_4 : Constant  Value=4  OutDataTypeStr=single
  desired_velocity : Constant  Value=4  OutDataTypeStr=single
  desired_voltage : Constant  Value=4  OutDataTypeStr=single
  ena_verbose : Constant  Value=false  OutDataTypeStr=boolean
  entlr : Constant  Value=0  OutDataTypeStr=uint8
  has_hall : Constant  Value=true  OutDataTypeStr=boolean
  has_qe : Constant  Value=true  OutDataTypeStr=boolean
  has_speed_qe : Constant  Value=false  OutDataTypeStr=boolean
  has_tsens : Constant  Value=false  OutDataTypeStr=boolean
  motor : Constant  Value=true  OutDataTypeStr=boolean
  motor_bool : Constant  Value=true  OutDataTypeStr=boolean
  nominal : Constant  Value=0  OutDataTypeStr=single
  peak : Constant  Value=0  OutDataTypeStr=single
  poles : Constant  Value=7  OutDataTypeStr=uint8
  rotencres : Constant  Value=16000  OutDataTypeStr=int16
  rotindexoff : Constant  Value=0  OutDataTypeStr=int16
  use_index : Constant  Value=true  OutDataTypeStr=boolean
  Out1 : Outport
  wires:
  desired_current_4/1 -> Bus Creator3/1  "desired_current"
  motor_bool/1 -> Bus Creator/1, Bus Creator4/1  "motor"
  Bus Creator3/1 -> Bus Creator1/3  "BUS_MSG_DESIRED_TARGETS"
  Bus Creator2/1 -> Bus Creator1/1  "BUS_MSG_CONTROL_MODE"
  motor/1 -> Bus Creator2/1  "motor"
  Bus Creator/1 -> Bus Creator1/4
  Kp_4/1 -> Bus Creator/2
  Ki_4/1 -> Bus Creator/3
  peak/1 -> Bus Creator4/3  "peak"
  nominal/1 -> Bus Creator4/2  "nominal"
  Bus Creator4/1 -> Bus Creator1/2  "BUS_MSG_CURRENT_LIMIT"
  Overcurrent_4/1 -> Bus Creator4/4
  Ks_4/1 -> Bus Creator/5
  Kd_4/1 -> Bus Creator/4
  ControlMode_4/1 -> Bus Creator2/2  "control_mode"
  Bus Creator1/1 -> Out1/1
  has_speed_qe/1 -> Bus Creator5/3
  has_hall/1 -> Bus Creator5/1
  rotindexoff/1 -> Bus Creator5/10
  entlr/1 -> Bus Creator5/8
  has_tsens/1 -> Bus Creator5/4
  rotencres/1 -> Bus Creator5/9
  poles/1 -> Bus Creator5/7
  ena_verbose/1 -> Bus Creator5/6
  has_qe/1 -> Bus Creator5/2
  use_index/1 -> Bus Creator5/5
  Bus Creator5/1 -> Bus Creator1/5
  desired_voltage/1 -> Bus Creator3/2  "desired_current"
  desired_velocity/1 -> Bus Creator3/3  "desired_current"
